simulink model "single_phase_inverter"  (R2026a)
settings: Solver=ode23tb  StopTime=param.sim.simlength  FixedStep=tc  MaxStep=param.glb_time.tc
values from neighbouring files (symbols this model uses):
  param = add_template_extras(param, options)    [init_model.m]
libraries: fl_lib x45, nesl_utility x24, single_phase_transformer_lib x3, phase_shift_filter x2, phase_shift_filter_ccaller x2, three_phase_voltage_with_frt_emulator x1, power_meter_iec x1, single_phase_transformer x1, three_phase_diode_rectifier x1, three_phase_diode_rectifier_with_thermal_model x1, full_bridge_ideal_switch x1, full_bridge_mosfet_based_with_thermal_model x1
(part 2 of 4)

== system single_phase_inverter/grid/grid_emulator/threephase_vi_measures ==
  Bus Creator : BusCreator  Inputs=6
  Current Sensor : fl_lib/Electrical/Electrical Sensors/Current Sensor
  Current Sensor1 : fl_lib/Electrical/Electrical Sensors/Current Sensor
  Current Sensor2 : fl_lib/Electrical/Electrical Sensors/Current Sensor
  Electrical Reference1 : fl_lib/Electrical/Electrical Elements/Electrical Reference
  Voltage Sensor : fl_lib/Electrical/Electrical Sensors/Voltage Sensor
  Voltage Sensor1 : fl_lib/Electrical/Electrical Sensors/Voltage Sensor
  Voltage Sensor2 : fl_lib/Electrical/Electrical Sensors/Voltage Sensor
  i : Selector  InputPortWidth=6  IndexOptions=Index vector (dialog)  Indices=[4 5 6]  OutputSizes=1
  ia_grid : nesl_utility/PS-Simulink Converter  PhysicalDomain=network_engine_domain  SubClassName=ps_output  LeftPortType=input  RightPortType=output  PseudoPeriodic=off  Frequencies=[]  VectorFormat=1-D array  Unit=A  AffineConversion=off
  ib_grid : nesl_utility/PS-Simulink Converter  PhysicalDomain=network_engine_domain  SubClassName=ps_output  LeftPortType=input  RightPortType=output  PseudoPeriodic=off  Frequencies=[]  VectorFormat=1-D array  Unit=A  AffineConversion=off
  ic_grid : nesl_utility/PS-Simulink Converter  PhysicalDomain=network_engine_domain  SubClassName=ps_output  LeftPortType=input  RightPortType=output  PseudoPeriodic=off  Frequencies=[]  VectorFormat=1-D array  Unit=A  AffineConversion=off
  u : Selector  InputPortWidth=6  IndexOptions=Index vector (dialog)  Indices=[1 2 3]  OutputSizes=1
  ua_grid : nesl_utility/PS-Simulink Converter  PhysicalDomain=network_engine_domain  SubClassName=ps_output  LeftPortType=input  RightPortType=output  PseudoPeriodic=off  Frequencies=[]  VectorFormat=1-D array  Unit=V  AffineConversion=off
  ub_grid : nesl_utility/PS-Simulink Converter  PhysicalDomain=network_engine_domain  SubClassName=ps_output  LeftPortType=input  RightPortType=output  PseudoPeriodic=off  Frequencies=[]  VectorFormat=1-D array  Unit=V  AffineConversion=off
  uc_grid : nesl_utility/PS-Simulink Converter  PhysicalDomain=network_engine_domain  SubClassName=ps_output  LeftPortType=input  RightPortType=output  PseudoPeriodic=off  Frequencies=[]  VectorFormat=1-D array  Unit=V  AffineConversion=off
  Ua : PMIOPort  Side=Left
  ua : PMIOPort  Port=2  Side=Right
  Ub : PMIOPort  Port=3  Side=Left
  ub : PMIOPort  Port=4  Side=Right
  Uc : PMIOPort  Port=5  Side=Left
  uc : PMIOPort  Port=6  Side=Right
  tag scope: i_abc_line=global, u_abc_line=global
  wires:
  Bus Creator/1 -> i/1, u/1  "vi_data"
  ib_grid/1 -> Bus Creator/5  "ib"
  ia_grid/1 -> Bus Creator/4  "ia"
  ic_grid/1 -> Bus Creator/6  "ic"
  ua_grid/1 -> Bus Creator/1  "ua"
  ub_grid/1 -> Bus Creator/2  "ub"
  uc_grid/1 -> Bus Creator/3  "uc"
  i/1 -> [i_abc_line]
  u/1 -> [u_abc_line]
  connections:
  Current Sensor1/LConn1 -- Ub/RConn1 -- Voltage Sensor1/LConn1
  Electrical Reference1/LConn1 -- Voltage Sensor/RConn2 -- Voltage Sensor2/RConn2 -- Voltage Sensor1/RConn2
  Voltage Sensor/RConn1 -- ua_grid/LConn1
  Current Sensor/RConn2 -- ua/RConn1
  Voltage Sensor1/RConn1 -- ub_grid/LConn1
  Voltage Sensor2/LConn1 -- Current Sensor2/LConn1 -- Uc/RConn1
  Current Sensor/LConn1 -- Ua/RConn1 -- Voltage Sensor/LConn1
  Current Sensor1/RConn2 -- ub/RConn1
  Voltage Sensor2/RConn1 -- uc_grid/LConn1
  ib_grid/LConn1 -- Current Sensor1/RConn1
  ia_grid/LConn1 -- Current Sensor/RConn1
  ic_grid/LConn1 -- Current Sensor2/RConn1
  Current Sensor2/RConn2 -- uc/RConn1

== system single_phase_inverter/single_phase_inverter/single phase inverter/full_bridge_ideal_switch_based ==
  gate_commands : Inport
  full-bridge ideal switch based : full_bridge_ideal_switch/full-bridge ideal switch based  Rds_on=1.85e-3  Vdon_diode=0.35  Rdon_diode=1.85e-3  Csnubber=6e-9  Rsnubber=3e3  Vth=7.5
  uac(+) : PMIOPort  Side=Right
  udc(+) : PMIOPort  Port=2  Side=Left
  uac(-) : PMIOPort  Port=3  Side=Right
  udc(-) : PMIOPort  Port=4  Side=Left
  tag scope: full_bridge_ideal_switch_data=global
  wires:
  full-bridge ideal switch based/1 -> [full_bridge_ideal_switch_data]
  gate_commands/1 -> full-bridge ideal switch based/1
  connections:
  full-bridge ideal switch based/RConn1 -- uac(+)/RConn1
  udc(-)/RConn1 -- full-bridge ideal switch based/LConn2
  udc(+)/RConn1 -- full-bridge ideal switch based/LConn1
  full-bridge ideal switch based/RConn2 -- uac(-)/RConn1

== system single_phase_inverter/single_phase_inverter/single phase inverter/full_bridge_mosfet_based_with_thermal_model ==
  gate_commands : Inport
  Bus Selector : BusSelector  OutputSignals=mosfet_ploss_Q1,mosfet_voltage_Q1,mosfet_current_Q1,mosfet_JH_temp_Q1,mosfet_HA_temp_Q1
  Bus Selector1 : BusSelector  OutputSignals=mosfet_ploss_Q2,mosfet_voltage_Q2,mosfet_current_Q2,mosfet_JH_temp_Q2,mosfet_HA_temp_Q2
  full-bridge mosfet based with thermal model : full_bridge_mosfet_based_with_thermal_model/full-bridge mosfet based with thermal model  mass_heatsink_m=param.thermal.heatsink.no_weight  specific_heat_m=param.thermal.heatsink.cp  rth_mosfet_HA_m=param.thermal.heatsink.Rth_mosfet_HA  rth_mosfet_JH_m=param.spinv.mosfet.Rth_mosfet_JH  Rds_on_m=param.spinv.mosfet.Rds_on  Vth_m=param.spinv.mosfet.Vth  Eon_m=param.spinv.mosfet.Eon  Eoff_m=param.spinv.mosfet.Eoff  Voff_sw_loss_m=param.spinv.mosfet.Voff_sw_losses  Ion_sw_loss_m=param.spinv.mosfet.Ion_sw_losses  Vdon_diode_m=param.spinv.mosfet.Vdon_diode  Rdon_diode_m=param.spinv.mosfet.Rdon_diode  JunctionTermalMass_m=param.spinv.mosfet.JunctionTermalMass  Tambient_m=param.thermal.heatsink.Tambient  DThs_init_m=param.thermal.heatsink.DThs_init
  udc(+) : PMIOPort  Side=Left
  uac(+) : PMIOPort  Port=2  Side=Right
  udc(-) : PMIOPort  Port=3  Side=Left
  uac(-) : PMIOPort  Port=4  Side=Right
  tag scope: full_bridge_mosfet_data=global, mosfet_HA_temp_invQ1=global, mosfet_HA_temp_invQ2=global, mosfet_JH_temp_invQ1=global, mosfet_JH_temp_invQ2=global, mosfet_current_invQ1=global, mosfet_current_invQ2=global, mosfet_ploss_invQ1=global, mosfet_ploss_invQ2=global, mosfet_voltage_invQ1=global, mosfet_voltage_invQ2=global
  wires:
  Bus Selector/1 -> [mosfet_ploss_invQ1]  "<mosfet_ploss_Q1>"
  Bus Selector1/3 -> [mosfet_current_invQ2]  "<mosfet_current_Q2>"
  Bus Selector/2 -> [mosfet_voltage_invQ1]  "<mosfet_voltage_Q1>"
  Bus Selector1/4 -> [mosfet_JH_temp_invQ2]  "<mosfet_JH_temp_Q2>"
  Bus Selector1/1 -> [mosfet_ploss_invQ2]  "<mosfet_ploss_Q2>"
  Bus Selector1/5 -> [mosfet_HA_temp_invQ2]  "<mosfet_HA_temp_Q2>"
  Bus Selector/4 -> [mosfet_JH_temp_invQ1]  "<mosfet_JH_temp_Q1>"
  Bus Selector/3 -> [mosfet_current_invQ1]  "<mosfet_current_Q1>"
  Bus Selector1/2 -> [mosfet_voltage_invQ2]  "<mosfet_voltage_Q2>"
  full-bridge mosfet based with thermal model/1 -> [full_bridge_mosfet_data], Bus Selector1/1, Bus Selector/1
  Bus Selector/5 -> [mosfet_HA_temp_invQ1]  "<mosfet_HA_temp_Q1>"
  gate_commands/1 -> full-bridge mosfet based with thermal model/1
  connections:
  full-bridge mosfet based with thermal model/LConn2 -- udc(-)/RConn1
  full-bridge mosfet based with thermal model/LConn1 -- udc(+)/RConn1
  full-bridge mosfet based with thermal model/RConn1 -- uac(+)/RConn1
  full-bridge mosfet based with thermal model/RConn2 -- uac(-)/RConn1

== system single_phase_inverter/single_phase_inverter/single phase inverter control/acquisition_and_scaling_current ==
  in : Inport
  1/Ti5 : Gain  Gain=1/param.spinv.hw.ibez  SaturateOnIntegerOverflow=on  OutDataTypeStr=Inherit: Same as input  ParamDataTypeStr=Inherit: Same as input
  Quantizer : Quantizer  QuantizationInterval=param.meas.adc_quantization
  out : Outport
  wires:
  Quantizer/1 -> out/1
  1/Ti5/1 -> Quantizer/1
  in/1 -> 1/Ti5/1

== system single_phase_inverter/single_phase_inverter/single phase inverter control/acquisition_and_scaling_current_with_white_noise ==
  in : Inport
  1/Ti5 : Gain  Gain=1/param.spinv.hw.ibez  SaturateOnIntegerOverflow=on  OutDataTypeStr=Inherit: Same as input  ParamDataTypeStr=Inherit: Same as input
  Band-Limited White Noise : simulink/Sources/Band-Limited White Noise  Commented=on  Cov=1e-10  Ts=param.glb_time.tc  seed=[23341]
  Quantizer : Quantizer  QuantizationInterval=param.meas.adc12_quantization
  Sum : Sum  Inputs=|++
  current_measure_with-without noise : Scope  NumInputPorts=2
      settings: ActiveDisplayYMinimum=-1.259685411609524  ActiveDisplayYMaximum=1.2603394332468927  DataLoggingVariableName=ScopeData15
  out : Outport
  wires:
  in/1 -> 1/Ti5/1
  1/Ti5/1 -> Sum/1, current_measure_with-without noise/1  "iload_without_noise"
  Sum/1 -> Quantizer/1
  Band-Limited White Noise/1 -> Sum/2
  Quantizer/1 -> out/1, current_measure_with-without noise/2  "iload_with_noise"

== system single_phase_inverter/single_phase_inverter/single phase inverter control/acquisition_and_scaling_dc_voltage ==
  in : Inport
  1/Ti3 : Gain  Gain=1/param.spinv.hw.udc_nom  SaturateOnIntegerOverflow=on  OutDataTypeStr=Inherit: Same as input  ParamDataTypeStr=Inherit: Same as input
  Quantizer : Quantizer  QuantizationInterval=param.meas.adc12_quantization
  out : Outport
  wires:
  in/1 -> 1/Ti3/1
  1/Ti3/1 -> Quantizer/1
  Quantizer/1 -> out/1

== system single_phase_inverter/single_phase_inverter/single phase inverter control/acquisition_and_scaling_grid_voltage_ac ==
  in : Inport
  1/Ti5 : Gain  Gain=1/param.grid.emu.u2bez  SaturateOnIntegerOverflow=on  OutDataTypeStr=Inherit: Same as input  ParamDataTypeStr=Inherit: Same as input
  Quantizer : Quantizer  QuantizationInterval=param.meas.adc12_quantization
  out : Outport
  wires:
  Quantizer/1 -> out/1
  1/Ti5/1 -> Quantizer/1
  in/1 -> 1/Ti5/1

== system single_phase_inverter/single_phase_inverter/single phase inverter control/acquisition_and_scaling_voltage ==
  in : Inport
  1/Ti5 : Gain  Gain=1/param.spinv.hw.ubez  SaturateOnIntegerOverflow=on  OutDataTypeStr=Inherit: Same as input  ParamDataTypeStr=Inherit: Same as input
  Quantizer : Quantizer  QuantizationInterval=param.meas.adc12_quantization
  pwm filtering for measure : cstblocks_lti/LTI System  sys=param.spinv.sogi.flt.beta  IC=[]  PadeOrder=0
  out : Outport
  wires:
  in/1 -> 1/Ti5/1
  pwm filtering for measure/1 -> Quantizer/1
  1/Ti5/1 -> pwm filtering for measure/1
  Quantizer/1 -> out/1

== system single_phase_inverter/single_phase_inverter/single phase inverter control/inverter_current_output_pu_reference ==
  Gain : Gain
  Rate Limiter : RateLimiter  RisingSlewLimit=param.grid.emu.omega_grid_nom  FallingSlewLimit=-param.grid.emu.omega_grid_nom  SampleTimeMode=inherited
  Sum : Sum  Inputs=+++
  i_out_inverter_reference_step1 : Step  Time=param.spinv.ref.time_step_ref_1  FinalValue=param.spinv.ref.iph_grid_pu_ref_1  SampleTime=0
  i_out_inverter_reference_step2 : Step  Time=param.spinv.ref.time_step_ref_2  FinalValue=param.spinv.ref.iph_grid_pu_ref_2  SampleTime=0
  i_out_inverter_reference_step3 : Step  Time=param.spinv.ref.time_step_ref_3  FinalValue=param.spinv.ref.iph_grid_pu_ref_3  SampleTime=0
  inverter_current_output_pu_reference : Outport
  wires:
  Rate Limiter/1 -> Gain/1
  Sum/1 -> Rate Limiter/1
  Gain/1 -> inverter_current_output_pu_reference/1
  i_out_inverter_reference_step1/1 -> Sum/2
  i_out_inverter_reference_step2/1 -> Sum/3
  i_out_inverter_reference_step3/1 -> Sum/1

== system single_phase_inverter/single_phase_inverter/single phase inverter control/pwm modulator ==
  vout : Inport
  Constant : Constant  Value=0
  Single phase two level PWM generator with global TRGO : single_phase_pwm_modulator/Single phase two level PWM generator with global TRGO  f=param.glb_time.fPWM_INV  m_up=0.98  m_low=0.02  dead_time=param.glb_time.dead_time_INV  pos_cmd_gate=18  neg_cmd_gate=-3  polarity=-1  tc=param.glb_time.tc  double_sampling=param.glb_time.TRGO_INV_double_update
  gate_cmds : Outport
  tag scope: TRGO_INV_1=global
  wires:
  vout/1 -> Single phase two level PWM generator with global TRGO/3
  Constant/1 -> Single phase two level PWM generator with global TRGO/2
  Single phase two level PWM generator with global TRGO/2 -> gate_cmds/1
  Single phase two level PWM generator with global TRGO/1 -> [TRGO_INV_1]
  [time_inv_module_1] -> Single phase two level PWM generator with global TRGO/1

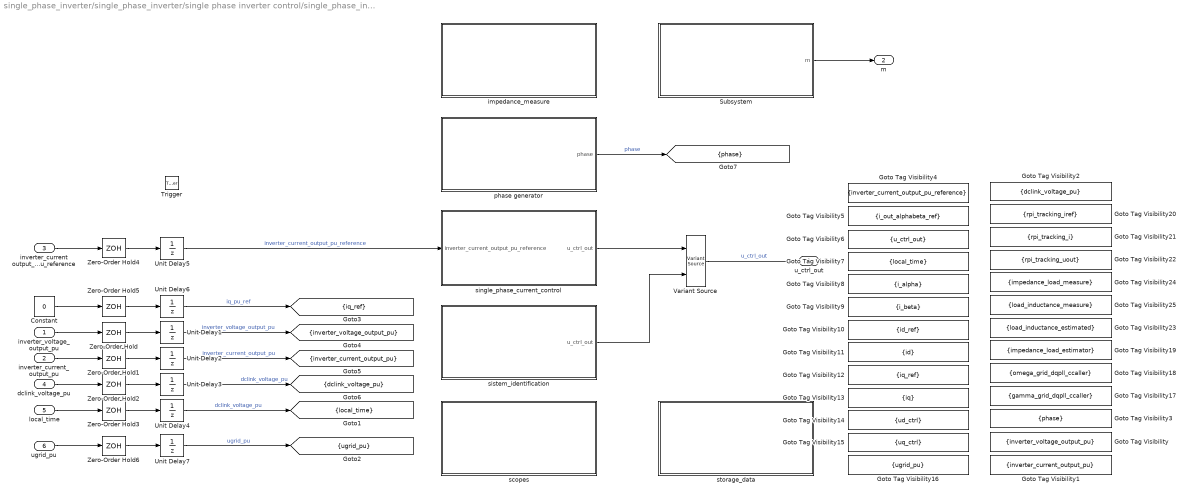
== system single_phase_inverter/single_phase_inverter/single phase inverter control/single_phase_inverter_ctrl ==
  inverter_voltage_output_pu : Inport
  inverter_current_output_pu : Inport  Port=2
  inverter_current output_pu_reference : Inport  Port=3
  dclink_voltage_pu : Inport  Port=4
  local_time : Inport  Port=5
  ugrid_pu : Inport  Port=6
  Trigger : TriggerPort  VariantControl=(inherit)  PortDimensions=1
  Constant : Constant  Value=0
  Goto Tag Visibility : GotoTagVisibility  GotoTag=inverter_voltage_output_pu
  Goto Tag Visibility1 : GotoTagVisibility  GotoTag=inverter_current_output_pu
  Goto Tag Visibility10 : GotoTagVisibility  GotoTag=id_ref
  Goto Tag Visibility11 : GotoTagVisibility  GotoTag=id
  Goto Tag Visibility12 : GotoTagVisibility  GotoTag=iq_ref
  Goto Tag Visibility13 : GotoTagVisibility  GotoTag=iq
  Goto Tag Visibility14 : GotoTagVisibility  GotoTag=ud_ctrl
  Goto Tag Visibility15 : GotoTagVisibility  GotoTag=uq_ctrl
  Goto Tag Visibility16 : GotoTagVisibility  GotoTag=ugrid_pu
  Goto Tag Visibility17 : GotoTagVisibility  GotoTag=gamma_grid_dqpll_ccaller
  Goto Tag Visibility18 : GotoTagVisibility  GotoTag=omega_grid_dqpll_ccaller
  Goto Tag Visibility19 : GotoTagVisibility  GotoTag=impedance_load_estimator
  Goto Tag Visibility2 : GotoTagVisibility  GotoTag=dclink_voltage_pu
  Goto Tag Visibility20 : GotoTagVisibility  GotoTag=rpi_tracking_iref
  Goto Tag Visibility21 : GotoTagVisibility  GotoTag=rpi_tracking_i
  Goto Tag Visibility22 : GotoTagVisibility  GotoTag=rpi_tracking_uout
  Goto Tag Visibility23 : GotoTagVisibility  GotoTag=load_inductance_estimated
  Goto Tag Visibility24 : GotoTagVisibility  GotoTag=impedance_load_measure
  Goto Tag Visibility25 : GotoTagVisibility  GotoTag=load_inductance_measure
  Goto Tag Visibility3 : GotoTagVisibility  GotoTag=phase
  Goto Tag Visibility4 : GotoTagVisibility  GotoTag=inverter_current_output_pu_reference
  Goto Tag Visibility5 : GotoTagVisibility  GotoTag=i_out_alphabeta_ref
  Goto Tag Visibility6 : GotoTagVisibility  GotoTag=u_ctrl_out
  Goto Tag Visibility7 : GotoTagVisibility  GotoTag=local_time
  Goto Tag Visibility8 : GotoTagVisibility  GotoTag=i_alpha
  Goto Tag Visibility9 : GotoTagVisibility  GotoTag=i_beta
  Subsystem : Subsystem
  Unit Delay{1..7} (7 alike) : UnitDelay  SampleTime=-1
  Variant Source : VariantSource  VariantControls={param.spinv.system_identification_enable == 0, param.spinv.system_identification_enable == 1}
  Zero-Order Hold{,1..6} (7 alike) : ZeroOrderHold  SampleTime=-1
  impedance_measure : Subsystem
  phase generator : Subsystem
  scopes : Subsystem
  single_phase_current_control : Subsystem
  sistem_identification : Subsystem
  storage_data : Subsystem
  u_ctrl_out : Outport
  m : Outport  Port=2
  tag scope: dclink_voltage_pu=scoped, inverter_current_output_pu=scoped, inverter_voltage_output_pu=scoped, iq_ref=scoped, local_time=scoped, phase=scoped, ugrid_pu=scoped
  wires:
  inverter_voltage_output_pu/1 -> Zero-Order Hold/1
  inverter_current_output_pu/1 -> Zero-Order Hold1/1
  dclink_voltage_pu/1 -> Zero-Order Hold2/1
  Unit Delay1/1 -> [inverter_voltage_output_pu]  "inverter_voltage_output_pu"
  Unit Delay2/1 -> [inverter_current_output_pu]  "inverter_current_output_pu"
  Unit Delay3/1 -> [dclink_voltage_pu]  "dclink_voltage_pu"
  phase generator/1(phase) -> [phase]  "phase"
  inverter_current output_pu_reference/1 -> Zero-Order Hold4/1
  single_phase_current_control/1(u_ctrl_out) -> Variant Source/1
  Variant Source/1 -> u_ctrl_out/1  "u_ctrl_out"
  sistem_identification/1(u_ctrl_out) -> Variant Source/2
  Zero-Order Hold/1 -> Unit Delay1/1
  Zero-Order Hold1/1 -> Unit Delay2/1
  Zero-Order Hold2/1 -> Unit Delay3/1
  Zero-Order Hold3/1 -> Unit Delay4/1
  Unit Delay4/1 -> [local_time]  "dclink_voltage_pu"
  local_time/1 -> Zero-Order Hold3/1
  Zero-Order Hold4/1 -> Unit Delay5/1
  Unit Delay5/1 -> single_phase_current_control/1(inverter_current_output_pu_reference)  "inverter_current_output_pu_reference"
  Constant/1 -> Zero-Order Hold5/1
  Zero-Order Hold5/1 -> Unit Delay6/1
  Unit Delay6/1 -> [iq_ref]  "iq_pu_ref"
  ugrid_pu/1 -> Zero-Order Hold6/1
  Zero-Order Hold6/1 -> Unit Delay7/1
  Unit Delay7/1 -> [ugrid_pu]  "ugrid_pu"
  Subsystem/1(m) -> m/1

== system single_phase_inverter/single_phase_inverter/single phase inverter control/single_phase_inverter_ctrl/Subsystem ==
  Bus Creator : BusCreator  Inputs=21
  m : Outport
  wires:
  [i_out_alphabeta_ref] -> Bus Creator/4  "i_out_inverter_pu_ref"
  [rpi_tracking_iref] -> Bus Creator/16  "rpi_tracking_iref"
  [inverter_current_output_pu] -> Bus Creator/2  "inverter_current_output_pu"
  [iq] -> Bus Creator/12  "iq"
  [i_alpha] -> Bus Creator/7  "i_alpha"
  [uq_ctrl] -> Bus Creator/14  "uq_ctrl"
  [impedance_load_measure] -> Bus Creator/20  "impedance_load_measure"
  [ud_ctrl] -> Bus Creator/13  "ud_ctrl"
  [u_ctrl_out] -> Bus Creator/5  "u_ctrl_out"
  [inverter_voltage_output_pu] -> Bus Creator/1  "inverter_voltage_output_pu"
  [id_ref] -> Bus Creator/9  "id_ref"
  [local_time] -> Bus Creator/6  "local_time"
  [rpi_tracking_uout] -> Bus Creator/18  "rpi_tracking_uout"
  [rpi_tracking_i] -> Bus Creator/17  "rpi_tracking_i"
  [iq_ref] -> Bus Creator/11  "iq_ref"
  [i_beta] -> Bus Creator/8  "i_beta"
  [impedance_load_estimator] -> Bus Creator/15  "impedance_load_estimator"
  [id] -> Bus Creator/10  "id"
  [load_inductance_estimated] -> Bus Creator/19  "load_inductance_estimated"
  Bus Creator/1 -> m/1
  [inverter_current_output_pu_reference] -> Bus Creator/3  "inverter_current_output_pu_reference"
  [load_inductance_measure] -> Bus Creator/21  "load_inductance_measure"

== system single_phase_inverter/single_phase_inverter/single phase inverter control/single_phase_inverter_ctrl/impedance_measure ==
  Constant : Constant  Value=param.spinv.omega_set
  Gain1 : Gain  Gain=1/param.spinv.omega_set
  Product : Product  Inputs=*/*
  Saturation : Saturate  UpperLimit=inf  LowerLimit=0.05
  Saturation1 : Saturate  UpperLimit=inf  LowerLimit=0.05
  Subsystem : Subsystem
  dclink voltage pu : Scope
      settings: ActiveDisplayYMinimum=0.61963581267726608  ActiveDisplayYMaximum=0.99084450439297456  DataLoggingVariableName=ScopeData10
  dmavg_flt : moving_average_filter/dmavg_flt  ts=param.glb_time.ts_afe  enable_time=0.025
  load_measure : Scope  NumInputPorts=4
      settings: ActiveDisplayYMinimum=-0.14197120195714497  ActiveDisplayYMaximum=1.277740817614305  DataLoggingVariableName=ScopeData2
  module_iload : Subsystem
  module_uctrl_out : Subsystem
  tag scope: impedance_load_measure=scoped, load_inductance_measure=scoped
  wires:
  module_uctrl_out/1(u_ctrl) -> Product/1
  Saturation/1 -> Product/2
  module_iload/1(iload) -> Saturation/1  "Iload"
  [i_alpha] -> load_measure/3, module_iload/1(i_alpha)  "i_alpha_sogi"
  [i_beta] -> load_measure/4, module_iload/2(i_beta)  "i_beta_sogi"
  [uq_ctrl] -> module_uctrl_out/2(uq_ctrl)
  [ud_ctrl] -> module_uctrl_out/1(ud_ctrl)
  Constant/1 -> dmavg_flt/2
  dmavg_flt/1 -> Gain1/1, load_measure/1, [impedance_load_measure]  "Xload"
  Gain1/1 -> load_measure/2, [load_inductance_measure]  "Lload"
  [dclink_voltage_pu] -> Saturation1/1
  Saturation1/1 -> dclink voltage pu/1, Product/3
  Product/1 -> Subsystem/1(Xload)  "Xload"
  Subsystem/1(Xload1) -> dmavg_flt/1

== system single_phase_inverter/single_phase_inverter/single phase inverter control/single_phase_inverter_ctrl/phase generator ==
  Bus Creator : BusCreator  Inputs=3
  Bus Creator1 : BusCreator  Inputs=2
  Constant : Constant  Value=param.spinv.ctrl.omega_base
  Gain : Gain  Gain=param.glb_time.ts_inv
  Sum : Sum  Inputs=|++
  Unit Delay : UnitDelay  SampleTime=-1
  Variant Source : VariantSource  VariantControls={param.spinv.frequency_set ~= param.grid.emu.fgrid_nom, param.spinv.frequency_set == param.grid.emu.fgrid_nom}
  bounder1 : MATLAB Function  TreatAsAtomicUnit=on
  dq_pll_ccaller : Subsystem
  dqpll_ccaler : Scope  NumInputPorts=3
      settings: ActiveDisplayYMinimum=-3.89557489045133  ActiveDisplayYMaximum=3.8955748904514897  DataLoggingVariableName=ScopeData3
  phase : Outport
  tag scope: gamma_grid_dqpll_ccaller=scoped, omega_grid_dqpll_ccaller=scoped
  wires:
  Sum/1 -> Unit Delay/1
  Constant/1 -> Gain/1
  Unit Delay/1 -> bounder1/1(u)
  Gain/1 -> Sum/1
  bounder1/1(y) -> Sum/2, Variant Source/1  "phase"
  dq_pll_ccaller/4(dqpll_ueta) -> Bus Creator/2  "ueta_n"
  dq_pll_ccaller/3(dqpll_uxi) -> Bus Creator/1  "uxi_n"
  dq_pll_ccaller/1(gamma_hat) -> [gamma_grid_dqpll_ccaller]
  dq_pll_ccaller/2(omega_pu_hat) -> [omega_grid_dqpll_ccaller]
  dq_pll_ccaller/5(dqpll_state) -> Bus Creator/3  "dqpll_state"
  [ugrid_pu] -> dq_pll_ccaller/1(ug_abc_pu)
  [gamma_grid_dqpll_ccaller] -> Variant Source/2
  [gamma_grid_dqpll_ccaller] -> Bus Creator1/1  "gamma_grid_dqpll"
  [omega_grid_dqpll_ccaller] -> Bus Creator1/2  "omega_grid_dqpll"
  Bus Creator1/1 -> dqpll_ccaler/3
  Bus Creator/1 -> dqpll_ccaler/2
  Variant Source/1 -> dqpll_ccaler/1, phase/1  "phase_set"

== system single_phase_inverter/single_phase_inverter/single phase inverter control/single_phase_inverter_ctrl/scopes ==
  Bus Creator1 : BusCreator  Inputs=3
  Bus Creator2 : BusCreator  Inputs=2
  Bus Creator3 : BusCreator  Inputs=2
  Bus Creator4 : BusCreator  Inputs=2
  single phase inverter tracking current scope 1 : Scope  NumInputPorts=2
      settings: ActiveDisplayYMinimum=-1.23468017578125  ActiveDisplayYMaximum=1.23419189453125  DataLoggingVariableName=ScopeData12
  single phase inverter tracking current scope 2 : Scope  NumInputPorts=2
      settings: ActiveDisplayYMinimum=-1.2499947587050575  ActiveDisplayYMaximum=1.2499948046096099  DataLoggingVariableName=ScopeData2
  wires:
  Bus Creator1/1 -> single phase inverter tracking current scope 1/2  "is_tracking"
  [i_out_alphabeta_ref] -> Bus Creator1/2  "i_out_inverter_pu_ref"
  [inverter_current_output_pu] -> Bus Creator1/3  "inverter_current_output_pu"
  [inverter_voltage_output_pu] -> Bus Creator2/1  "inverter_voltage_output_pu"
  Bus Creator2/1 -> single phase inverter tracking current scope 1/1  "load"
  [inverter_current_output_pu_reference] -> Bus Creator1/1  "inverter_current_output_pu_reference"
  [inverter_current_output_pu] -> Bus Creator2/2  "inverter_current_output_pu"
  [u_ctrl_out] -> Bus Creator3/1  "u_ctrl_out"
  [inverter_voltage_output_pu] -> Bus Creator3/2  "inverter_voltage_output_pu"
  Bus Creator3/1 -> single phase inverter tracking current scope 2/2  "u_load"
  [inverter_current_output_pu] -> Bus Creator4/2  "inverter_current_output_pu"
  [i_out_alphabeta_ref] -> Bus Creator4/1  "i_out_alphabeta_ref"
  Bus Creator4/1 -> single phase inverter tracking current scope 2/1  "i_load"

== system single_phase_inverter/single_phase_inverter/single phase inverter control/single_phase_inverter_ctrl/single_phase_current_control ==
  inverter_current_output_pu_reference : Inport
  Variant Source : VariantSource  VariantControls={param.spinv.rpi_enable == 1, param.spinv.rpi_enable == 0}
  current_reference_generation : Subsystem
  dqpi_current_controller : Subsystem
  rpi_current_controller : Subsystem
  u_ctrl_out : Outport
  tag scope: i_out_alphabeta_ref=scoped, inverter_current_output_pu_reference=scoped, u_ctrl_out=scoped
  wires:
  rpi_current_controller/1(u_ctrl_out) -> Variant Source/1  "u_ctrl_out"
  dqpi_current_controller/1(u_out) -> Variant Source/2  "u_ctrl_out"
  current_reference_generation/1(is_ref) -> [i_out_alphabeta_ref], rpi_current_controller/1(i_ref)  "i_out_inverter_pu_ref"
  Variant Source/1 -> u_ctrl_out/1, [u_ctrl_out]  "u_ctrl_out"
  [phase] -> current_reference_generation/2(phase)
  inverter_current_output_pu_reference/1 -> current_reference_generation/1(mag_ref), [inverter_current_output_pu_reference]
  current_reference_generation/2(id_ref) -> dqpi_current_controller/1(id_ref)

== system single_phase_inverter/single_phase_inverter/single phase inverter control/single_phase_inverter_ctrl/sistem_identification ==
  open loop u/f : Subsystem
  u_ctrl_out : Outport
  wires:
  open loop u/f/1(u_out) -> u_ctrl_out/1  "u_ctrl_out"

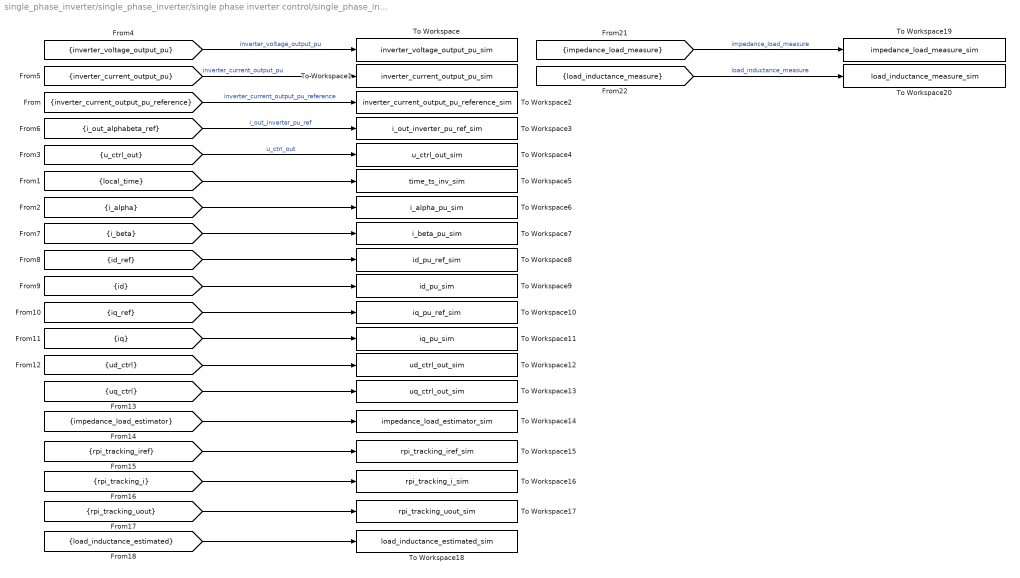
== system single_phase_inverter/single_phase_inverter/single phase inverter control/single_phase_inverter_ctrl/storage_data ==
  To Workspace : ToWorkspace  VariableName=inverter_voltage_output_pu_sim  SampleTime=-1
      settings: MaxDataPoints=param.glb_time.Ns_inv  Save2DSignal=2-D array (concatenate along first dimension)
  To Workspace1 : ToWorkspace  VariableName=inverter_current_output_pu_sim  SampleTime=-1
      settings: MaxDataPoints=param.glb_time.Ns_inv  Save2DSignal=2-D array (concatenate along first dimension)
  To Workspace10 : ToWorkspace  VariableName=iq_pu_ref_sim  SampleTime=-1
      settings: MaxDataPoints=param.glb_time.Ns_inv  Save2DSignal=2-D array (concatenate along first dimension)
  To Workspace11 : ToWorkspace  VariableName=iq_pu_sim  SampleTime=-1
      settings: MaxDataPoints=param.glb_time.Ns_inv  Save2DSignal=2-D array (concatenate along first dimension)
  To Workspace12 : ToWorkspace  VariableName=ud_ctrl_out_sim  SampleTime=-1
      settings: MaxDataPoints=param.glb_time.Ns_inv  Save2DSignal=2-D array (concatenate along first dimension)
  To Workspace13 : ToWorkspace  VariableName=uq_ctrl_out_sim  SampleTime=-1
      settings: MaxDataPoints=param.glb_time.Ns_inv  Save2DSignal=2-D array (concatenate along first dimension)
  To Workspace14 : ToWorkspace  VariableName=impedance_load_estimator_sim  SampleTime=-1
      settings: MaxDataPoints=param.glb_time.Ns_inv  Save2DSignal=2-D array (concatenate along first dimension)
  To Workspace15 : ToWorkspace  VariableName=rpi_tracking_iref_sim  SampleTime=-1
      settings: MaxDataPoints=param.glb_time.Ns_inv  Save2DSignal=2-D array (concatenate along first dimension)
  To Workspace16 : ToWorkspace  VariableName=rpi_tracking_i_sim  SampleTime=-1
      settings: MaxDataPoints=param.glb_time.Ns_inv  Save2DSignal=2-D array (concatenate along first dimension)
  To Workspace17 : ToWorkspace  VariableName=rpi_tracking_uout_sim  SampleTime=-1
      settings: MaxDataPoints=param.glb_time.Ns_inv  Save2DSignal=2-D array (concatenate along first dimension)
  To Workspace18 : ToWorkspace  VariableName=load_inductance_estimated_sim  SampleTime=-1
      settings: MaxDataPoints=param.glb_time.Ns_inv  Save2DSignal=2-D array (concatenate along first dimension)
  To Workspace19 : ToWorkspace  VariableName=impedance_load_measure_sim  SampleTime=-1
      settings: MaxDataPoints=param.glb_time.Ns_inv  Save2DSignal=2-D array (concatenate along first dimension)
  To Workspace2 : ToWorkspace  VariableName=inverter_current_output_pu_reference_sim  SampleTime=-1
      settings: MaxDataPoints=param.glb_time.Ns_inv  Save2DSignal=2-D array (concatenate along first dimension)
  To Workspace20 : ToWorkspace  VariableName=load_inductance_measure_sim  SampleTime=-1
      settings: MaxDataPoints=param.glb_time.Ns_inv  Save2DSignal=2-D array (concatenate along first dimension)
  To Workspace3 : ToWorkspace  VariableName=i_out_inverter_pu_ref_sim  SampleTime=-1
      settings: MaxDataPoints=param.glb_time.Ns_inv  Save2DSignal=2-D array (concatenate along first dimension)
  To Workspace4 : ToWorkspace  VariableName=u_ctrl_out_sim  SampleTime=-1
      settings: MaxDataPoints=param.glb_time.Ns_inv  Save2DSignal=2-D array (concatenate along first dimension)
  To Workspace5 : ToWorkspace  VariableName=time_ts_inv_sim  SampleTime=-1
      settings: MaxDataPoints=param.glb_time.Ns_inv  Save2DSignal=2-D array (concatenate along first dimension)
  To Workspace6 : ToWorkspace  VariableName=i_alpha_pu_sim  SampleTime=-1
      settings: MaxDataPoints=param.glb_time.Ns_inv  Save2DSignal=2-D array (concatenate along first dimension)
  To Workspace7 : ToWorkspace  VariableName=i_beta_pu_sim  SampleTime=-1
      settings: MaxDataPoints=param.glb_time.Ns_inv  Save2DSignal=2-D array (concatenate along first dimension)
  To Workspace8 : ToWorkspace  VariableName=id_pu_ref_sim  SampleTime=-1
      settings: MaxDataPoints=param.glb_time.Ns_inv  Save2DSignal=2-D array (concatenate along first dimension)
  To Workspace9 : ToWorkspace  VariableName=id_pu_sim  SampleTime=-1
      settings: MaxDataPoints=param.glb_time.Ns_inv  Save2DSignal=2-D array (concatenate along first dimension)
  wires:
  [inverter_voltage_output_pu] -> To Workspace/1  "inverter_voltage_output_pu"
  [inverter_current_output_pu] -> To Workspace1/1  "inverter_current_output_pu"
  [inverter_current_output_pu_reference] -> To Workspace2/1  "inverter_current_output_pu_reference"
  [i_out_alphabeta_ref] -> To Workspace3/1  "i_out_inverter_pu_ref"
  [u_ctrl_out] -> To Workspace4/1  "u_ctrl_out"
  [local_time] -> To Workspace5/1
  [i_alpha] -> To Workspace6/1
  [i_beta] -> To Workspace7/1
  [id_ref] -> To Workspace8/1
  [id] -> To Workspace9/1
  [iq_ref] -> To Workspace10/1
  [iq] -> To Workspace11/1
  [ud_ctrl] -> To Workspace12/1
  [uq_ctrl] -> To Workspace13/1
  [impedance_load_estimator] -> To Workspace14/1
  [rpi_tracking_iref] -> To Workspace15/1
  [rpi_tracking_i] -> To Workspace16/1
  [rpi_tracking_uout] -> To Workspace17/1
  [load_inductance_estimated] -> To Workspace18/1
  [load_inductance_measure] -> To Workspace20/1  "load_inductance_measure"
  [impedance_load_measure] -> To Workspace19/1  "impedance_load_measure"

== system single_phase_inverter/single_phase_inverter/single phase inverter control/single_phase_inverter_ctrl/impedance_measure/Subsystem ==
  Xload : Inport
  Constant : Constant  Value=param.spinv.hw.udc_nom
  Constant1 : Constant  Value=param.spinv.hw.ibez
  Constant2 : Constant  Value=param.spinv.hw.norm.Xbez
  MATLAB Function : MATLAB Function  TreatAsAtomicUnit=on
  Xload1 : Outport
  wires:
  MATLAB Function/1(y) -> Xload1/1  "Xload"
  Xload/1 -> MATLAB Function/1(u)
  Constant/1 -> MATLAB Function/2(Vdc_FS)
  Constant1/1 -> MATLAB Function/3(Vac_FS)
  Constant2/1 -> MATLAB Function/4(Xbez)

== system single_phase_inverter/single_phase_inverter/single phase inverter control/single_phase_inverter_ctrl/impedance_measure/module_iload ==
  i_alpha : Inport
  i_beta : Inport  Port=2
  Sqrt : Sqrt
  Square : Math  Operator=square
  Square1 : Math  Operator=square
  Sum : Sum  Inputs=|++
  iload : Outport
  wires:
  i_beta/1 -> Square1/1
  i_alpha/1 -> Square/1
  Square/1 -> Sum/1
  Sum/1 -> Sqrt/1
  Square1/1 -> Sum/2
  Sqrt/1 -> iload/1

== system single_phase_inverter/single_phase_inverter/single phase inverter control/single_phase_inverter_ctrl/impedance_measure/module_uctrl_out ==
  ud_ctrl : Inport
  uq_ctrl : Inport  Port=2
  Sqrt : Sqrt
  Square : Math  Operator=square
  Square1 : Math  Operator=square
  Sum : Sum  Inputs=|++
  u_ctrl : Outport
  wires:
  Sqrt/1 -> u_ctrl/1
  Square1/1 -> Sum/2
  Sum/1 -> Sqrt/1
  Square/1 -> Sum/1
  ud_ctrl/1 -> Square/1
  uq_ctrl/1 -> Square1/1

== system single_phase_inverter/single_phase_inverter/single phase inverter control/single_phase_inverter_ctrl/phase generator/dq_pll_ccaller ==
  ug_abc_pu : Inport
  Constant : Constant  Value=param.glb_time.ts_inv
  Demux : Demux  Outputs=3
  Step : Step  Time=0.01  InitialValue=1  FinalValue=0
  dqpll_grid_ccaller : Subsystem
  first_harmonic_tracker : Scope  NumInputPorts=3
      settings: ActiveDisplayYMinimum=-1.3190075680613518  ActiveDisplayYMaximum=1.2165602371096611
  first_harmonic_tracker1 : Subsystem
  first_harmonic_tracker2 : Subsystem
  first_harmonic_tracker3 : Subsystem
  gamma_hat : Outport  VectorParamsAs1DForOutWhenUnconnected=off
  omega_pu_hat : Outport  Port=2  VectorParamsAs1DForOutWhenUnconnected=off
  dqpll_uxi : Outport  Port=3  VectorParamsAs1DForOutWhenUnconnected=off
  dqpll_ueta : Outport  Port=4  VectorParamsAs1DForOutWhenUnconnected=off
  dqpll_state : Outport  Port=5  VectorParamsAs1DForOutWhenUnconnected=off
  wires:
  ug_abc_pu/1 -> Demux/1
  Demux/1 -> first_harmonic_tracker1/1(u)
  Demux/2 -> first_harmonic_tracker2/1(u)
  Demux/3 -> first_harmonic_tracker3/1(u)
  first_harmonic_tracker1/1(u_hat) -> first_harmonic_tracker/1, dqpll_grid_ccaller/2(phase_u)  "tracker_phase_u"
  first_harmonic_tracker2/1(u_hat) -> first_harmonic_tracker/2, dqpll_grid_ccaller/3(phase_v)  "tracker_phase_v"
  first_harmonic_tracker3/1(u_hat) -> first_harmonic_tracker/3, dqpll_grid_ccaller/4(phase_w)  "tracker_phase_w"
  Step/1 -> dqpll_grid_ccaller/1(reset)
  Constant/1 -> dqpll_grid_ccaller/5(ts)
  dqpll_grid_ccaller/1(gamma_hat) -> gamma_hat/1
  dqpll_grid_ccaller/2(omega_pu_hat) -> omega_pu_hat/1
  dqpll_grid_ccaller/3(dqpll_uxi) -> dqpll_uxi/1
  dqpll_grid_ccaller/4(dqpll_ueta) -> dqpll_ueta/1
  dqpll_grid_ccaller/5(dqpll_state) -> dqpll_state/1

== system single_phase_inverter/single_phase_inverter/single phase inverter control/single_phase_inverter_ctrl/single_phase_current_control/current_reference_generation ==
  mag_ref : Inport
  phase : Inport  Port=2
  Bus Creator : BusCreator  Inputs=2
  Product : Product
  Product1 : Product
  Sin : Trigonometry  Operator=cos
  Sin1 : Trigonometry
  is_ref : Outport
  id_ref : Outport  Port=2
  wires:
  Sin/1 -> Product/2
  phase/1 -> Sin1/1, Sin/1
  mag_ref/1 -> id_ref/1, Product1/1, Product/1
  Sin1/1 -> Product1/2
  Product/1 -> Bus Creator/1  "is_ref_alpha"
  Product1/1 -> Bus Creator/2  "is_ref_beta"
  Bus Creator/1 -> is_ref/1

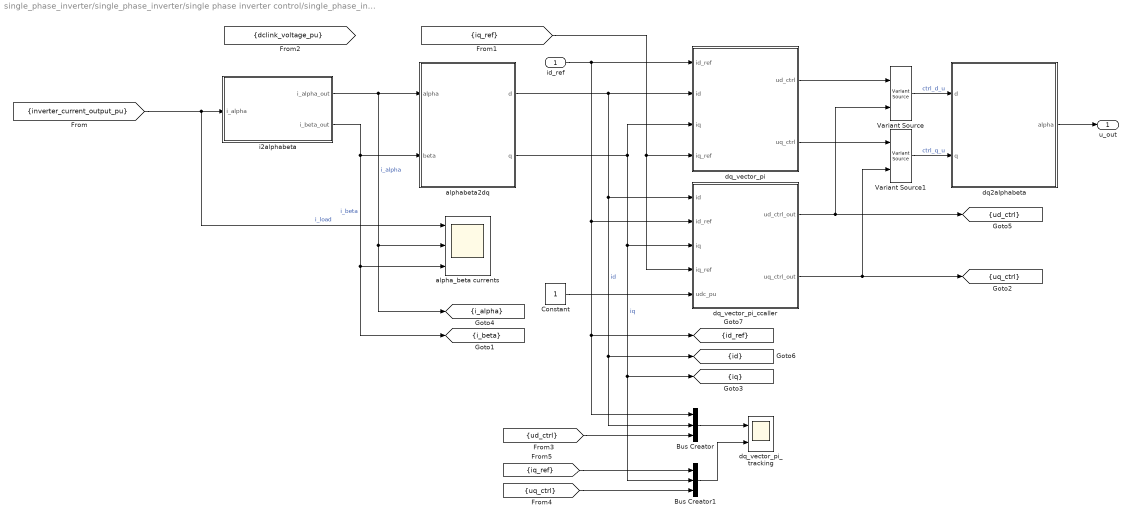
== system single_phase_inverter/single_phase_inverter/single phase inverter control/single_phase_inverter_ctrl/single_phase_current_control/dqpi_current_controller ==
  id_ref : Inport
  Bus Creator : BusCreator  Inputs=3
  Bus Creator1 : BusCreator  Inputs=3
  Constant : Constant
  Variant Source : VariantSource  VariantControls={param.spinv.impl.use_current_controller_from_ccaller_mod1 == 0, param.spinv.impl.use_current_controller_from_ccaller_mod1 == 1}
  Variant Source1 : VariantSource  VariantControls={param.spinv.impl.use_current_controller_from_ccaller_mod1 == 0, param.spinv.impl.use_current_controller_from_ccaller_mod1 == 1}
  alpha_beta currents : Scope  NumInputPorts=3
      settings: ActiveDisplayYMinimum=-1.351318359375  ActiveDisplayYMaximum=1.326904296875  DataLoggingVariableName=ScopeData2
  alphabeta2dq : Subsystem
  dq2alphabeta : Subsystem
  dq_vector_pi : Subsystem
  dq_vector_pi_ccaller : Subsystem
  dq_vector_pi_tracking : Scope  NumInputPorts=2
      settings: ActiveDisplayYMinimum=-0.17788174446714192  ActiveDisplayYMaximum=0.16687413354305455  DataLoggingVariableName=ScopeData8
  i2alphabeta : Subsystem
  u_out : Outport
  tag scope: i_alpha=scoped, i_beta=scoped, id=scoped, id_ref=scoped, iq=scoped, ud_ctrl=scoped, uq_ctrl=scoped
  wires:
  dq2alphabeta/1(alpha) -> u_out/1
  id_ref/1 -> dq_vector_pi/1(id_ref), Bus Creator/1, [id_ref], dq_vector_pi_ccaller/2(id_ref)
  alphabeta2dq/1("d ") -> Bus Creator/2, [id], dq_vector_pi_ccaller/1(id), dq_vector_pi/2(id)  "id"
  alphabeta2dq/2("q ") -> dq_vector_pi/3(iq), Bus Creator1/2, [iq], dq_vector_pi_ccaller/3(iq)  "iq"
  [iq_ref] -> dq_vector_pi/4(iq_ref), dq_vector_pi_ccaller/4(iq_ref)
  Variant Source1/1 -> dq2alphabeta/2(q)  "ctrl_q_u"
  Variant Source/1 -> dq2alphabeta/1(d)  "ctrl_d_u"
  dq_vector_pi/1(ud_ctrl) -> Variant Source/1
  dq_vector_pi/2(uq_ctrl) -> Variant Source1/1
  Constant/1 -> dq_vector_pi_ccaller/5(udc_pu)
  dq_vector_pi_ccaller/1(ud_ctrl_out) -> [ud_ctrl], Variant Source/2
  dq_vector_pi_ccaller/2(uq_ctrl_out) -> [uq_ctrl], Variant Source1/2
  Bus Creator1/1 -> dq_vector_pi_tracking/2
  Bus Creator/1 -> dq_vector_pi_tracking/1
  [ud_ctrl] -> Bus Creator/3
  [uq_ctrl] -> Bus Creator1/3
  [iq_ref] -> Bus Creator1/1
  [inverter_current_output_pu] -> alpha_beta currents/1, i2alphabeta/1(i_alpha)  "i_load"
  i2alphabeta/1(i_alpha_out) -> alpha_beta currents/2, [i_alpha], alphabeta2dq/1(alpha)  "i_alpha"
  i2alphabeta/2(i_beta_out) -> [i_beta], alpha_beta currents/3, alphabeta2dq/2(beta)  "i_beta"

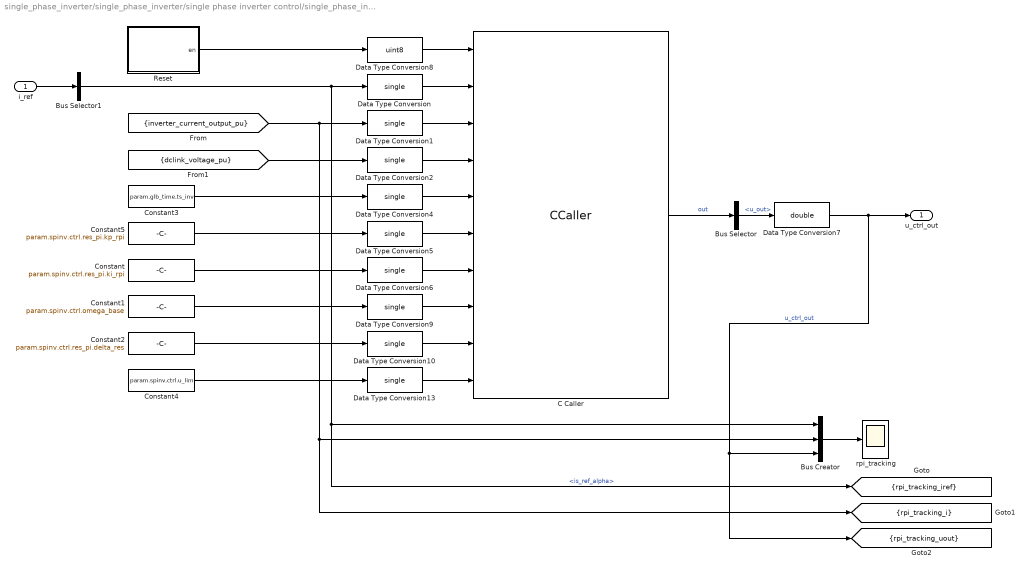
== system single_phase_inverter/single_phase_inverter/single phase inverter control/single_phase_inverter_ctrl/single_phase_current_control/rpi_current_controller ==
  i_ref : Inport
  Bus Creator : BusCreator  Inputs=3
  Bus Selector : BusSelector  OutputSignals=u_out
  Bus Selector1 : BusSelector  OutputSignals=is_ref_alpha
  C Caller : CCaller  FunctionName=rpi_process_simulink  PortSpecificationStruct="%)30     .    V!(   8    (     @         %    \"     L    !     0         %  0 \"0    $    _    07)G3F%M90  4&]R=$YA;64 4V-O<&4     26YD97@     5'EP90      4VEZ90      27-';&]B86P   X    P    !@    @    $          4    (     0    ,    !         !   P!O=70 #@   #     &    \"     0         !0    @    !     P    $         $  # &]U=  .    .     8    (    !          %    \"     $    &     0         0   ...(+6126 chars)"
  Constant : Constant  Value=param.spinv.ctrl.res_pi.ki_rpi
  Constant1 : Constant  Value=param.spinv.ctrl.omega_base
  Constant2 : Constant  Value=param.spinv.ctrl.res_pi.delta_res
  Constant3 : Constant  Value=param.glb_time.ts_inv
  Constant4 : Constant  Value=param.spinv.ctrl.u_lim
  Constant5 : Constant  Value=param.spinv.ctrl.res_pi.kp_rpi
  Data Type Conversion{,1..2,4..6,9..10,13} (9 alike) : DataTypeConversion  OutDataTypeStr=single  SaturateOnIntegerOverflow=off  RndMeth=Floor
  Data Type Conversion7 : DataTypeConversion  OutDataTypeStr=double  SaturateOnIntegerOverflow=off  RndMeth=Floor
  Data Type Conversion8 : DataTypeConversion  OutDataTypeStr=uint8  SaturateOnIntegerOverflow=off  RndMeth=Floor
  Reset : Subsystem
  rpi_tracking : Scope
      settings: ActiveDisplayYMinimum=-3.0104694962501526  ActiveDisplayYMaximum=2.1558924317359924  DataLoggingVariableName=ScopeData14
  u_ctrl_out : Outport
  tag scope: rpi_tracking_i=scoped, rpi_tracking_iref=scoped, rpi_tracking_uout=scoped
  wires:
  Constant4/1 -> Data Type Conversion13/1
  Constant2/1 -> Data Type Conversion10/1
  Constant1/1 -> Data Type Conversion9/1
  Constant/1 -> Data Type Conversion6/1
  Data Type Conversion8/1 -> C Caller/1
  Data Type Conversion/1 -> C Caller/2
  Data Type Conversion1/1 -> C Caller/3
  Data Type Conversion2/1 -> C Caller/4
  Data Type Conversion4/1 -> C Caller/5
  Data Type Conversion5/1 -> C Caller/6
  Data Type Conversion6/1 -> C Caller/7
  Data Type Conversion9/1 -> C Caller/8
  Data Type Conversion10/1 -> C Caller/9
  Data Type Conversion13/1 -> C Caller/10
  Constant3/1 -> Data Type Conversion4/1
  Constant5/1 -> Data Type Conversion5/1
  [dclink_voltage_pu] -> Data Type Conversion2/1
  [inverter_current_output_pu] -> [rpi_tracking_i], Bus Creator/2, Data Type Conversion1/1
  i_ref/1 -> Bus Selector1/1
  Reset/1(en) -> Data Type Conversion8/1
  C Caller/1 -> Bus Selector/1  "out"
  Bus Selector/1 -> Data Type Conversion7/1  "<u_out>"
  Bus Selector1/1 -> [rpi_tracking_iref], Bus Creator/1, Data Type Conversion/1  "<is_ref_alpha>"
  Bus Creator/1 -> rpi_tracking/1
  Data Type Conversion7/1 -> u_ctrl_out/1, [rpi_tracking_uout], Bus Creator/3  "u_ctrl_out"

== system single_phase_inverter/single_phase_inverter/single phase inverter control/single_phase_inverter_ctrl/sistem_identification/open loop u//f ==
  Constant2 : Constant  Value=0.35
  Data Store Memory : DataStoreMemory  DataStoreName=u_test  WriteAfterWriteMsg=warning  ShowAdditionalParam=off
  Data Store Read1 : DataStoreRead  DataStoreName=u_test  DataStoreElements=u_test  IndexOptions=Index vector (dialog)  Indices=1  OutputSizes=1
  Data Store Write : DataStoreWrite  DataStoreName=u_test  IndexOptions=Index vector (dialog)  Indices=1  OutputSizes=1
  Gain1 : Gain  Gain=1/param.spinv.omega_set
  Gain2 : Gain  Gain=param.spinv.hw.udc_bez/param.spinv.hw.ubez
  Gain3 : Gain  Gain=param.spinv.hw.ubez/param.spinv.hw.ibez
  Product : Product  Inputs=*/
  Saturation : Saturate  UpperLimit=inf  LowerLimit=0.1
  dq2alphabeta : Subsystem
  i2alphabeta : Subsystem
  i_alpha_beta_system_identification : Scope  NumInputPorts=4
      settings: ActiveDisplayYMinimum=-0.047392215508018642  ActiveDisplayYMaximum=3.1217734669527113  DataLoggingVariableName=ScopeData2
  module : Subsystem
  u_out : Outport
  tag scope: impedance_load_estimator=scoped, load_inductance_estimated=scoped
  wires:
  [inverter_current_output_pu] -> i2alphabeta/1(i_alpha)  "i_alpha"
  dq2alphabeta/1(alpha) -> u_out/1
  Data Store Read1/1 -> Product/1
  Constant2/1 -> Data Store Write/1
  Saturation/1 -> Product/2
  module/1(i) -> Saturation/1  "Iload"
  Gain1/1 -> [load_inductance_estimated], i_alpha_beta_system_identification/2  "Lload"
  i2alphabeta/1(i_alpha_out) -> i_alpha_beta_system_identification/3, module/1(i_alpha)  "i_alpha_sogi"
  i2alphabeta/2(i_beta_out) -> i_alpha_beta_system_identification/4, module/2(i_beta)  "i_beta_sogi"
  Product/1 -> Gain2/1
  Gain3/1 -> [impedance_load_estimator], i_alpha_beta_system_identification/1, Gain1/1  "Xload"
  Gain2/1 -> Gain3/1
